simulink model "normal"  (R2020a)
settings: Solver=ode45  StartTime=0.0  StopTime=0.4  FixedStep=1e-6  MaxStep=0.04  RelTol=1e-3  EnableMultiTasking=on
PreLoadFcn:
  | power_13NodeTestFeeder_init;
values from neighbouring files (symbols this model uses):
  C_601 = [1.03835973183e-08  -3.28956213337e-09  -2.07596127216e-09; -3.28956213337e-09  9.8230300863e-09  -1.22250137004e-09; -2.07596127216e-09  -1.22250137004e-09  9.29377945947e-09]    [Finalmat.mat]    (also in bus1.mat; bus10.mat; bus11.mat; bus12.mat)
  C_602 = [9.39333329896e-09  -1.78290377777e-09  -2.78635373607e-09; -1.78290377777e-09  8.5370713848e-09  -1.08586207709e-09; -2.78635373607e-09  -1.08586207709e-09  8.94105559107e-09]    [Finalmat.mat]    (also in bus1.mat; bus10.mat; bus11.mat; bus12.mat)
  C_603 = [0  0  0; 0  7.76272711671e-09  -1.48325331387e-09; 0  -1.48325331387e-09  7.69036927641e-09]    [Finalmat.mat]    (also in bus1.mat; bus10.mat; bus11.mat; bus12.mat)
  C_604 = [7.69036927641e-09  0  -1.48325331387e-09; 0  0  0; -1.48325331387e-09  0  7.76272711671e-09]    [Finalmat.mat]    (also in bus1.mat; bus10.mat; bus11.mat; bus12.mat)
  C_605 = [0  0  0; 0  0  0; 0  0  7.44890176838e-09]    [Finalmat.mat]    (also in bus1.mat; bus10.mat; bus11.mat; bus12.mat)
  C_606 = [1.59697709306e-07  -1.64824237567e-15  -1.64824237567e-15; -1.64824237567e-15  1.59697709306e-07  -1.64824237567e-15; -1.64824237567e-15  -1.64824237567e-15  1.59697709306e-07]    [Finalmat.mat]    (also in bus1.mat; bus10.mat; bus11.mat; bus12.mat)
  C_607 = [1.46679066902e-07  0  0; 0  0  0; 0  0  0]    [Finalmat.mat]    (also in bus1.mat; bus10.mat; bus11.mat; bus12.mat)
  ft2km = 0.0003048    [Finalmat.mat]    (also in bus1.mat; bus10.mat; bus11.mat; bus12.mat)
  L_601 = [0.0016777459142  0.000826923199875  0.000698195470335; 0.000826923199875  0.00172702836123  0.000634408490396; 0.000698195470335  0.000634408490396  0.00170560121035]    [Finalmat.mat]    (also in bus1.mat; bus10.mat; bus11.mat; bus12.mat)
  L_602 = [0.00194723354262  0.000698195470335  0.000826923199875; 0.000698195470335  0.00197508883877  0.000634408490396; 0.000826923199875  0.000634408490396  0.00199635116541]    [Finalmat.mat]    (also in bus1.mat; bus10.mat; bus11.mat; bus12.mat)
  L_603 = [0  0  0; 0  0.00222034730427  0.000756708074671; 0  0.000756708074671  0.00223650007955]    [Finalmat.mat]    (also in bus1.mat; bus10.mat; bus11.mat; bus12.mat)
  L_604 = [0.00223650007955  0  0.000756708074671; 0  0  0; 0.000756708074671  0  0.00222034730427]    [Finalmat.mat]    (also in bus1.mat; bus10.mat; bus11.mat; bus12.mat)
  L_605 = [0  0  0; 0  0  0; 0  0  0.00222100660122]    [Finalmat.mat]    (also in bus1.mat; bus10.mat; bus11.mat; bus12.mat)
  L_606 = [0.000735610572263  5.40623499221e-05  2.35698659721e-05; 5.40623499221e-05  0.000666054744009  5.40623499221e-05; 2.35698659721e-05  5.40623499221e-05  0.000735610572263]    [Finalmat.mat]    (also in bus1.mat; bus10.mat; bus11.mat; bus12.mat)
  L_607 = [0.000844559393295  0  0; 0  0  0; 0  0  0]    [Finalmat.mat]    (also in bus1.mat; bus10.mat; bus11.mat; bus12.mat)
  R_601 = [0.215305653249  0.0969341469174  0.0981768923907; 0.0969341469174  0.209713298619  0.0953807150757; 0.0981768923907  0.0953807150757  0.212136652292]    [Finalmat.mat]    (also in bus1.mat; bus10.mat; bus11.mat; bus12.mat)
  R_602 = [0.467645121603  0.0981768923907  0.0969341469174; 0.0981768923907  0.464476120646  0.0953807150757; 0.0969341469174  0.0953807150757  0.462052766973]    [Finalmat.mat]    (also in bus1.mat; bus10.mat; bus11.mat; bus12.mat)
  R_603 = [0  0  0; 0  0.826052916102  0.128375607392; 0  0.128375607392  0.822573228777]    [Finalmat.mat]    (also in bus1.mat; bus10.mat; bus11.mat; bus12.mat)
  R_604 = [0.822573228777  0  0.128375607392; 0  0  0; 0.128375607392  0  0.826052916102]    [Finalmat.mat]    (also in bus1.mat; bus10.mat; bus11.mat; bus12.mat)
  R_605 = [0  0  0; 0  0  0; 0  0  0.825928641555]    [Finalmat.mat]    (also in bus1.mat; bus10.mat; bus11.mat; bus12.mat)
  R_606 = [0.495979718394  0.198342177539  0.177029092672; 0.198342177539  0.49032522649  0.198342177539; 0.177029092672  0.198342177539  0.495979718394]    [Finalmat.mat]    (also in bus1.mat; bus10.mat; bus11.mat; bus12.mat)
  R_607 = [0.834192898952  0  0; 0  0  0; 0  0  0]    [Finalmat.mat]    (also in bus1.mat; bus10.mat; bus11.mat; bus12.mat)
libraries: neural x322, powerlib x54, powerlib_meascontrol x6, simulink x1
(part 2 of 8)

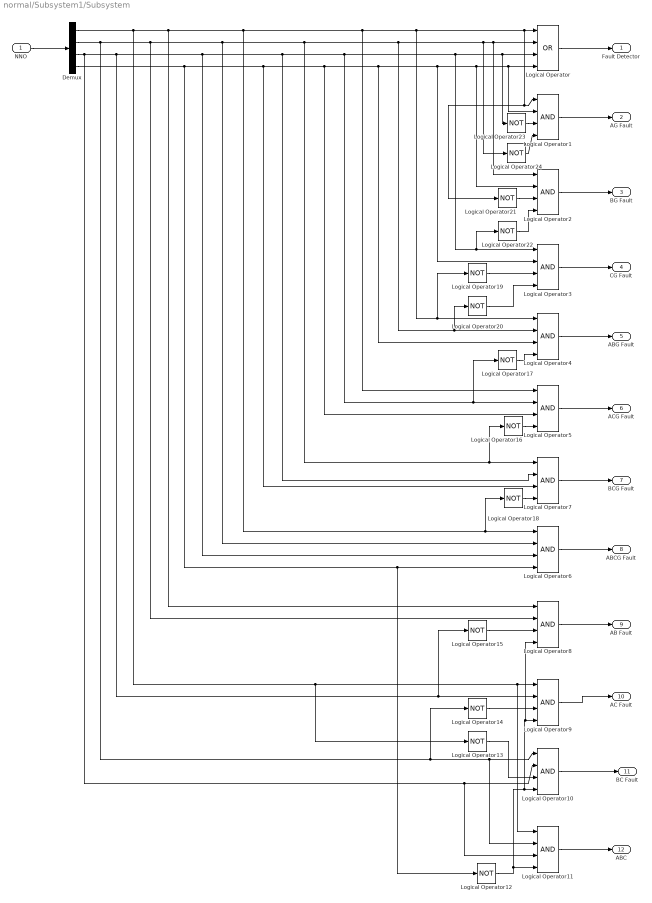
== system normal/Subsystem1/Subsystem ==
  NNO : Inport
  Demux : Demux
  Logical Operator : Logic  Operator=OR  Inputs=4  AllPortsSameDT=off  OutDataTypeStr=boolean
  Logical Operator{1..11} (11 alike) : Logic  Inputs=4  AllPortsSameDT=off  OutDataTypeStr=boolean
  Logical Operator{12..24} (13 alike) : Logic  Operator=NOT  AllPortsSameDT=off  OutDataTypeStr=boolean
  Fault Detector : Outport  VectorParamsAs1DForOutWhenUnconnected=off
  AG Fault : Outport  Port=2  VectorParamsAs1DForOutWhenUnconnected=off
  BG Fault : Outport  Port=3  VectorParamsAs1DForOutWhenUnconnected=off
  CG Fault : Outport  Port=4  VectorParamsAs1DForOutWhenUnconnected=off
  ABG Fault : Outport  Port=5  VectorParamsAs1DForOutWhenUnconnected=off
  ACG Fault : Outport  Port=6  VectorParamsAs1DForOutWhenUnconnected=off
  BCG Fault : Outport  Port=7  VectorParamsAs1DForOutWhenUnconnected=off
  ABCG Fault : Outport  Port=8  VectorParamsAs1DForOutWhenUnconnected=off
  AB Fault : Outport  Port=9  VectorParamsAs1DForOutWhenUnconnected=off
  AC Fault : Outport  Port=10  VectorParamsAs1DForOutWhenUnconnected=off
  BC Fault : Outport  Port=11  VectorParamsAs1DForOutWhenUnconnected=off
  ABC : Outport  Port=12  VectorParamsAs1DForOutWhenUnconnected=off
  wires:
  Logical Operator/1 -> Fault Detector/1
  NNO/1 -> Demux/1
  Demux/3 -> Logical Operator23/1, Logical Operator/3, Logical Operator22/1, Logical Operator3/1, Logical Operator17/1, Logical Operator5/2, Logical Operator7/2, Logical Operator6/3, Logical Operator15/1, Logical Operator9/2, Logical Operator11/3, Logical Operator10/2
  Demux/2 -> Logical Operator24/1, Logical Operator/2, Logical Operator2/1, Logical Operator20/1, Logical Operator4/2, Logical Operator16/1, Logical Operator7/1, Logical Operator6/2, Logical Operator8/2, Logical Operator14/1, Logical Operator11/2, Logical Operator10/1
  Demux/1 -> Logical Operator21/1, Logical Operator1/1, Logical Operator/1, Logical Operator19/1, Logical Operator4/1, Logical Operator5/1, Logical Operator18/1, Logical Operator6/1, Logical Operator8/1, Logical Operator13/1, Logical Operator11/1, Logical Operator9/1
  Demux/4 -> Logical Operator/4, Logical Operator1/2, Logical Operator2/2, Logical Operator3/2, Logical Operator4/3, Logical Operator5/3, Logical Operator7/3, Logical Operator12/1, Logical Operator6/4
  Logical Operator1/1 -> AG Fault/1
  Logical Operator2/1 -> BG Fault/1
  Logical Operator3/1 -> CG Fault/1
  Logical Operator4/1 -> ABG Fault/1
  Logical Operator5/1 -> ACG Fault/1
  Logical Operator7/1 -> BCG Fault/1
  Logical Operator6/1 -> ABCG Fault/1
  Logical Operator8/1 -> AB Fault/1
  Logical Operator11/1 -> ABC/1
  Logical Operator9/1 -> AC Fault/1
  Logical Operator10/1 -> BC Fault/1
  Logical Operator12/1 -> Logical Operator8/4, Logical Operator9/4, Logical Operator10/4, Logical Operator11/4
  Logical Operator13/1 -> Logical Operator10/3
  Logical Operator14/1 -> Logical Operator9/3
  Logical Operator15/1 -> Logical Operator8/3
  Logical Operator16/1 -> Logical Operator5/4
  Logical Operator17/1 -> Logical Operator4/4
  Logical Operator18/1 -> Logical Operator7/4
  Logical Operator19/1 -> Logical Operator3/3
  Logical Operator20/1 -> Logical Operator3/4
  Logical Operator22/1 -> Logical Operator2/4
  Logical Operator21/1 -> Logical Operator2/3
  Logical Operator23/1 -> Logical Operator1/3
  Logical Operator24/1 -> Logical Operator1/4

== system normal/Subsystem1/Function Fitting Neural Network/Layer 1 ==
  "p{1}" : Inport  PortDimensions=9
      mask Display: e = 0.06;c1 = [120 230 180]/255;c2 = ([120 230 180]+0)/(256+128);c3 = ([120 230 180]+128)/(256+128);patch([0 1 1 0],[0 0 1 1],c1);patch([0 1 1 1-e 1-e 0+e],[0 0 1 1-e 0+e 0+e],c2);patch([0 0 1 1-e 0+e 0+e],[0 1 1 1-e 1-e 0+e],c3);plot([0 1 1 0 0],[0 0 1 1 0]);
  Delays 1 : Subsystem
      mask Display: e = 0.06;c1 = [120 150 230]/255;c2 = ([120 150 230]+0)/383;c3 = ([120 150 230]+128)/383;patch([0 1 1 0],[0 0 1 1],c1);patch([0 1 1 1-e 1-e 0+e],[0 0 1 1-e 0+e 0+e],c2);patch([0 0 1 1-e 0+e 0+e],[0 1 1 1-e 1-e 0+e],c3);plot([0 1 1 0 0],[0 0 1 1 0]);disp('0');
  "IW{1,1}" : Subsystem
      mask Display: e = 0.06;c1 = [120 150 230]/255;c2 = ([120 150 230]+0)/383;c3 = ([120 150 230]+128)/383;patch([0 1 1 0],[0 0 1 1],c1);patch([0 1 1 1-e 1-e 0+e],[0 0 1 1-e 0+e 0+e],c2);patch([0 0 1 1-e 0+e 0+e],[0 1 1 1-e 1-e 0+e],c3);plot([0 1 1 0 0],[0 0 1 1 0]);disp('W');
  "b{1}" : Constant  Value=[1.4836701472282800562396687382715754210948944091796875;-4.6362530895366180772043662727810442447662353515625;-2.263086429812827926610907525173388421535491943359375;-2.5111547747930824669992944109253585338592529296875;0.56155923627202886105891366241849027574062347412109375;1.0307087915031150071598631257074885070323944091796875;-2.0460695401025663642258223262615501880645751953125;2.198522686181526797355445523862726986408233642578125;3.139278861361955552666813673567958176136016845703125;-1.9377980756718702348706528937327675521373748779296875;1.93447975728411147855467788758687674999237060546875;-1.9964334154407457067037512388196773827075958251953125;1.811849934043773036052016323083080351352691650390625;6.35238326894225480145905748941004276275634765625;3.1235450167660996356744362856261432170867919921875;-1.443640549170277953550112215452827513217926025390625;1.903051229366258478847839796799235045909881591796875;1.4333494363031633600513714554836042225360870361328125;-1.7974223905719768357158727667410857975482940673828125;-1.3000791505200501863015460912720300257205963134765625;0.392746284772382381333954981528222560882568359375;-1.78500042653535739844983254442922770977020263671875;1.5169851828956930628322652410133741796016693115234375;1.3899196529326232063539237060467712581157684326171875;0.88142263857842573226974991484894417226314544677734375;1.1298077443202012570822034831508062779903411865234375;1.6602576721865756059770546926301904022693634033203125;1.223520547142563419384941880707629024982452392578125;-1.520268524491023232059205838595516979694366455078125;0.929306052241560820448285085149109363555908203125;0.7195182400574877679133578567416407167911529541015625;0.53584680856447641783546487204148434102535247802734375;-2.402562935457116299886592969414778053760528564453125;0.0090962459951229000798544888084506965242326259613037109375;3.78523511409148749606856654281727969646453857421875;-0.14178662349532833442111723343259654939174652099609375;-0.34916324318866764908619870766415260732173919677734375;-0.42829990541065343645499297053902409970760345458984375;1.0935762893525506900260779730160720646381378173828125;0.7933443401718462961724753768066875636577606201171875;-0.19596363861845167431141589986509643495082855224609375;-2.881071814469615244291844646795652806758880615234375;2.561797995207929279359859719988889992237091064453125;-0.54218651761972835867453568425844423472881317138671875;-2.65640312734315831022513521020300686359405517578125;0.446493577723002743606883768734405748546123504638671875;-0.17177045244666844237002578665851615369319915771484375;-0.45537132588368745000906301356735639274120330810546875;-0.295732407345984660285154177472577430307865142822265625;-0.7946266943011830452547883396618999540805816650390625;0.9019892031651222108479259986779652535915374755859375;-0.5924118385813235132530962800956331193447113037109375;0.8851509988800858597102205749251879751682281494140625;-1.032020499483159436948653819854371249675750732421875;0.048154807323418695463868033357357489876449108123779296875;-0.72862529927491959114149722154252231121063232421875;0.9210456908434763168003200917155481874942779541015625;-2.14382668683358534877925194450654089450836181640625;0.128247662536615181227972470878739841282367706298828125;0.7914028966542192566890889793285168707370758056640625;-2.100152108028215724999654412386007606983184814453125;-0.075866072480479385120588631252758204936981201171875;0.2336366489054485795495708089219988323748111724853515625;2.12112491398540026210639553028158843517303466796875;-0.64362822141550546373167662750347517430782318115234375;0.9649124469060008646437154311570338904857635498046875;-0.85346406017299869528613953661988489329814910888671875;-0.47601133976015630455691507449955679476261138916015625;0.2488827845882790879006307704912615008652210235595703125;-0.10602051256760088027153443590577808208763599395751953125;2.0229387007712755774946344899944961071014404296875;0.8915126324932642898346557558397762477397918701171875 ...(+1511 chars)]
      mask Display: e = 0.06;c1 = [120 150 230]/255;c2 = ([120 150 230]+0)/383;c3 = ([120 150 230]+128)/383;patch([0 1 1 0],[0 0 1 1],c1);patch([0 1 1 1-e 1-e 0+e],[0 0 1 1-e 0+e 0+e],c2);patch([0 0 1 1-e 0+e 0+e],[0 1 1 1-e 1-e 0+e],c3);plot([0 1 1 0 0],[0 0 1 1 0]);disp('b');
  netsum : Sum  Inputs=2  InputSameDT=on  SaturateOnIntegerOverflow=on  OutDataTypeStr=Inherit: Same as first input
      mask Display: e = 0.06;c1 = [120 150 230]/255;c2 = ([120 150 230]+0)/383;c3 = ([120 150 230]+128)/383;patch([0 1 1 0],[0 0 1 1],c1);patch([0 1 1 1-e 1-e 0+e],[0 0 1 1-e 0+e 0+e],c2);patch([0 0 1 1-e 0+e 0+e],[0 1 1 1-e 1-e 0+e],c3);plot([0 1 1 0 0],[0 0 1 1 0]);disp('+');
  tansig : neural/Transfer Functions/tansig
  "a{1}" : Outport  InitialOutput=[0;0;0;0;0;0;0;0;0;0;0;0;0;0;0;0;0;0;0;0;0;0;0;0;0;0;0;0;0;0;0;0;0;0;0;0;0;0;0;0;0;0;0;0;0;0;0;0;0;0;0;0;0;0;0;0;0;0;0;0;0;0;0;0;0;0;0;0;0;0;0;0;0;0;0;0;0;0;0;0;0;0;0;0;0;0;0;0;0;0;0;0;0;0;0;0;0;0;0;0]
      mask Display: e = 0.06;c1 = [120 230 180]/255;c2 = ([120 230 180]+0)/(256+128);c3 = ([120 230 180]+128)/(256+128);patch([0 1 1 0],[0 0 1 1],c1);patch([0 1 1 1-e 1-e 0+e],[0 0 1 1-e 0+e 0+e],c2);patch([0 0 1 1-e 0+e 0+e],[0 1 1 1-e 1-e 0+e],c3);plot([0 1 1 0 0],[0 0 1 1 0]);
  wires:
  "p{1}"/1 -> Delays 1/1("p{1}")
  Delays 1/1("pd{1,1}") -> "IW{1,1}"/1("pd{1,1}")
  "IW{1,1}"/1("iz{1,1}") -> netsum/1
  "b{1}"/1 -> netsum/2
  netsum/1 -> tansig/1
  tansig/1 -> "a{1}"/1

== system normal/Subsystem1/Function Fitting Neural Network/Layer 2 ==
  "a{1} " : Inport  PortDimensions=100
      mask Display: e = 0.06;c1 = [120 230 180]/255;c2 = ([120 230 180]+0)/(256+128);c3 = ([120 230 180]+128)/(256+128);patch([0 1 1 0],[0 0 1 1],c1);patch([0 1 1 1-e 1-e 0+e],[0 0 1 1-e 0+e 0+e],c2);patch([0 0 1 1-e 0+e 0+e],[0 1 1 1-e 1-e 0+e],c3);plot([0 1 1 0 0],[0 0 1 1 0]);
  Delays 1 : Subsystem
      mask Display: e = 0.06;c1 = [120 150 230]/255;c2 = ([120 150 230]+0)/383;c3 = ([120 150 230]+128)/383;patch([0 1 1 0],[0 0 1 1],c1);patch([0 1 1 1-e 1-e 0+e],[0 0 1 1-e 0+e 0+e],c2);patch([0 0 1 1-e 0+e 0+e],[0 1 1 1-e 1-e 0+e],c3);plot([0 1 1 0 0],[0 0 1 1 0]);disp('0');
  "LW{2,1}" : Subsystem
      mask Display: e = 0.06;c1 = [120 150 230]/255;c2 = ([120 150 230]+0)/383;c3 = ([120 150 230]+128)/383;patch([0 1 1 0],[0 0 1 1],c1);patch([0 1 1 1-e 1-e 0+e],[0 0 1 1-e 0+e 0+e],c2);patch([0 0 1 1-e 0+e 0+e],[0 1 1 1-e 1-e 0+e],c3);plot([0 1 1 0 0],[0 0 1 1 0]);disp('W');
  "b{2}" : Constant  Value=0.73666496147771398650405672015040181577205657958984375
      mask Display: e = 0.06;c1 = [120 150 230]/255;c2 = ([120 150 230]+0)/383;c3 = ([120 150 230]+128)/383;patch([0 1 1 0],[0 0 1 1],c1);patch([0 1 1 1-e 1-e 0+e],[0 0 1 1-e 0+e 0+e],c2);patch([0 0 1 1-e 0+e 0+e],[0 1 1 1-e 1-e 0+e],c3);plot([0 1 1 0 0],[0 0 1 1 0]);disp('b');
  netsum : Sum  Inputs=2  InputSameDT=on  SaturateOnIntegerOverflow=on  OutDataTypeStr=Inherit: Same as first input
      mask Display: e = 0.06;c1 = [120 150 230]/255;c2 = ([120 150 230]+0)/383;c3 = ([120 150 230]+128)/383;patch([0 1 1 0],[0 0 1 1],c1);patch([0 1 1 1-e 1-e 0+e],[0 0 1 1-e 0+e 0+e],c2);patch([0 0 1 1-e 0+e 0+e],[0 1 1 1-e 1-e 0+e],c3);plot([0 1 1 0 0],[0 0 1 1 0]);disp('+');
  purelin : neural/Transfer Functions/purelin
  "a{2}" : Outport  InitialOutput=0
      mask Display: e = 0.06;c1 = [120 230 180]/255;c2 = ([120 230 180]+0)/(256+128);c3 = ([120 230 180]+128)/(256+128);patch([0 1 1 0],[0 0 1 1],c1);patch([0 1 1 1-e 1-e 0+e],[0 0 1 1-e 0+e 0+e],c2);patch([0 0 1 1-e 0+e 0+e],[0 1 1 1-e 1-e 0+e],c3);plot([0 1 1 0 0],[0 0 1 1 0]);
  wires:
  "a{1} "/1 -> Delays 1/1("p{2}")
  Delays 1/1("pd{2,1}") -> "LW{2,1}"/1("ad{2,1}")
  "LW{2,1}"/1("lz{2,1}") -> netsum/1
  "b{2}"/1 -> netsum/2
  netsum/1 -> purelin/1
  purelin/1 -> "a{2}"/1

== system normal/Subsystem1/Function Fitting Neural Network/Process Input 1 ==
  x : Inport  PortDimensions=9
      mask Display: e = 0.06;c1 = [120 230 180]/255;c2 = ([120 230 180]+0)/(256+128);c3 = ([120 230 180]+128)/(256+128);patch([0 1 1 0],[0 0 1 1],c1);patch([0 1 1 1-e 1-e 0+e],[0 0 1 1-e 0+e 0+e],c2);patch([0 0 1 1-e 0+e 0+e],[0 1 1 1-e 1-e 0+e],c3);plot([0 1 1 0 0],[0 0 1 1 0]);
  mapminmax : neural/Processing Functions/mapminmax  xmin=[4.0361303012440723492204597278;2.7248060221038734596277208766;4.10876986009723044190877772053;11.7997395123970481023434331291;9.69147739713131528560552396812;3.46457612151836746861022220401;6.39593571872652155718697031261;4.28688363604756350611069137813;6.97687974683904688077973332838]  xmax=[1771.43499266887192788999527693;1794.0488976631054356403183192;1779.62314843343483516946434975;2484.57589134188310708850622177;2501.74066788909203751245513558;2464.12499617464936818578280509;15623.5974818944614526117220521;15525.5512130097831686725839972;13147.2305966597232327330857515]  ymin=-1  ymax=1
  p : Outport  PortDimensions=9
      mask Display: e = 0.06;c1 = [120 230 180]/255;c2 = ([120 230 180]+0)/(256+128);c3 = ([120 230 180]+128)/(256+128);patch([0 1 1 0],[0 0 1 1],c1);patch([0 1 1 1-e 1-e 0+e],[0 0 1 1-e 0+e 0+e],c2);patch([0 0 1 1-e 0+e 0+e],[0 1 1 1-e 1-e 0+e],c3);plot([0 1 1 0 0],[0 0 1 1 0]);
  wires:
  x/1 -> mapminmax/1
  mapminmax/1 -> p/1

== system normal/Subsystem1/Function Fitting Neural Network/Process Output 1 ==
  a : Inport  PortDimensions=1
      mask Display: e = 0.06;c1 = [120 230 180]/255;c2 = ([120 230 180]+0)/(256+128);c3 = ([120 230 180]+128)/(256+128);patch([0 1 1 0],[0 0 1 1],c1);patch([0 1 1 1-e 1-e 0+e],[0 0 1 1-e 0+e 0+e],c2);patch([0 0 1 1-e 0+e 0+e],[0 1 1 1-e 1-e 0+e],c3);plot([0 1 1 0 0],[0 0 1 1 0]);
  mapminmax_reverse : neural/Processing Functions/mapminmax_reverse  xmin=0  xmax=6920  ymin=-1  ymax=1
  y : Outport  PortDimensions=1
      mask Display: e = 0.06;c1 = [120 230 180]/255;c2 = ([120 230 180]+0)/(256+128);c3 = ([120 230 180]+128)/(256+128);patch([0 1 1 0],[0 0 1 1],c1);patch([0 1 1 1-e 1-e 0+e],[0 0 1 1-e 0+e 0+e],c2);patch([0 0 1 1-e 0+e 0+e],[0 1 1 1-e 1-e 0+e],c3);plot([0 1 1 0 0],[0 0 1 1 0]);
  wires:
  a/1 -> mapminmax_reverse/1
  mapminmax_reverse/1 -> y/1

== system normal/Subsystem1/Function Fitting Neural Network1/Layer 1 ==
  "p{1}" : Inport  PortDimensions=9
      mask Display: e = 0.06;c1 = [120 230 180]/255;c2 = ([120 230 180]+0)/(256+128);c3 = ([120 230 180]+128)/(256+128);patch([0 1 1 0],[0 0 1 1],c1);patch([0 1 1 1-e 1-e 0+e],[0 0 1 1-e 0+e 0+e],c2);patch([0 0 1 1-e 0+e 0+e],[0 1 1 1-e 1-e 0+e],c3);plot([0 1 1 0 0],[0 0 1 1 0]);
  Delays 1 : Subsystem
      mask Display: e = 0.06;c1 = [120 150 230]/255;c2 = ([120 150 230]+0)/383;c3 = ([120 150 230]+128)/383;patch([0 1 1 0],[0 0 1 1],c1);patch([0 1 1 1-e 1-e 0+e],[0 0 1 1-e 0+e 0+e],c2);patch([0 0 1 1-e 0+e 0+e],[0 1 1 1-e 1-e 0+e],c3);plot([0 1 1 0 0],[0 0 1 1 0]);disp('0');
  "IW{1,1}" : Subsystem
      mask Display: e = 0.06;c1 = [120 150 230]/255;c2 = ([120 150 230]+0)/383;c3 = ([120 150 230]+128)/383;patch([0 1 1 0],[0 0 1 1],c1);patch([0 1 1 1-e 1-e 0+e],[0 0 1 1-e 0+e 0+e],c2);patch([0 0 1 1-e 0+e 0+e],[0 1 1 1-e 1-e 0+e],c3);plot([0 1 1 0 0],[0 0 1 1 0]);disp('W');
  "b{1}" : Constant  Value=[-2.13037715805268224045221359119750559329986572265625;2.746628097332809215203042185748927295207977294921875;2.796820994036730123610823284252546727657318115234375;0.4379379172983457468859569416963495314121246337890625;3.19223672506301081597257507382892072200775146484375;2.32496861654698694366061317850835621356964111328125;4.96726265985274917369451941340230405330657958984375;-1.697889576240742659507532152929343283176422119140625;2.298342309252483506298858628724701702594757080078125;1.966788681545197814415359971462748944759368896484375;-1.6125818559296110077383445968735031783580780029296875;1.5932178234269305239223513126489706337451934814453125;2.128810638902830731922222184948623180389404296875;-1.8112450514425881831215292550041340291500091552734375;-1.5788526096734150083733538849628530442714691162109375;-1.7955601924814892367265883876825682818889617919921875;-1.5849459381517727596389022437506355345249176025390625;-1.239288634212896145214699572534300386905670166015625;1.7228555051975666945196508095250464975833892822265625;-1.91686706005321649826100838254205882549285888671875;1.136660428733942129753131666802801191806793212890625;1.6784310129253030563489801352261565625667572021484375;-1.2868677081393820049726173238013871014118194580078125;1.4370556408635486445035667202319018542766571044921875;-1.5666891013466555104827193645178340375423431396484375;0.9782525744571939352312028859159909188747406005859375;1.56716358617225726135302465991117060184478759765625;-1.6998176443286594494708197089494206011295318603515625;-1.5458464297808092169361771084368228912353515625;1.0272554098359225616121648272383026778697967529296875;-1.1686228030247203246716480862232856452465057373046875;1.2392503600146891340472166120889596641063690185546875;-1.189381954438957667008480711956508457660675048828125;0.75198983869119218059751119653810746967792510986328125;0.358705656692439978083797313956893049180507659912109375;-0.92787680539037664662060933551401831209659576416015625;0.92975961512061078284574477947899140417575836181640625;-1.6601127850120409590317649417556822299957275390625;0.6862163993559653452081192881450988352298736572265625;0.351615586023979964647168117153341881930828094482421875;-0.9718618814417145923556518027908168733119964599609375;0.3834890515686317780108538499916903674602508544921875;1.1866027668763285962683085017488338053226470947265625;0.1954793823718590506377523752234992571175098419189453125;9.717970888699387188580658403225243091583251953125;5.33150149385156968406818123185075819492340087890625;0.47179814055236024561423846535035409033298492431640625;1.04948464890701931295780013897456228733062744140625;-0.95703425531130914549748922581784427165985107421875;0.1182206558537874097059017231003963388502597808837890625;0.150928108369996094584308821140439249575138092041015625;1.4935520252605691826630618379567749798297882080078125;-0.1574597910620717244878363771931617520749568939208984375;-0.493842571590737244857649557161494158208370208740234375;-0.1422139229762254541977739563662908039987087249755859375;-1.1294062657578962660664956274558790028095245361328125;6.2652904988000432950911999796517193317413330078125;-0.165122232426719417475169393583200871944427490234375;-0.7390589492982815311705735439318232238292694091796875;2.2778886380741969475138830603100359439849853515625;-0.2308917333994849607758936826940043829381465911865234375;0.171927231209594688632336101363762281835079193115234375;-0.69931808506733739161376206538989208638668060302734375;-0.43528701845326567276828200192539952695369720458984375;-1.708972287139544743439500962267629802227020263671875;-1.1665184635571332893988483192515559494495391845703125;1.14387762923370939205369722913019359111785888671875;1.48052201410643835544078683597035706043243408203125;-2.107332378231126401857409291551448404788970947265625;-3.493579865692837405077852963586337864398956298828125;1.414814221395528814895214964053593575954437255859375;0.06447901910621141319257532131814514286816120147705078125 ...(+1519 chars)]
      mask Display: e = 0.06;c1 = [120 150 230]/255;c2 = ([120 150 230]+0)/383;c3 = ([120 150 230]+128)/383;patch([0 1 1 0],[0 0 1 1],c1);patch([0 1 1 1-e 1-e 0+e],[0 0 1 1-e 0+e 0+e],c2);patch([0 0 1 1-e 0+e 0+e],[0 1 1 1-e 1-e 0+e],c3);plot([0 1 1 0 0],[0 0 1 1 0]);disp('b');
  netsum : Sum  Inputs=2  InputSameDT=on  SaturateOnIntegerOverflow=on  OutDataTypeStr=Inherit: Same as first input
      mask Display: e = 0.06;c1 = [120 150 230]/255;c2 = ([120 150 230]+0)/383;c3 = ([120 150 230]+128)/383;patch([0 1 1 0],[0 0 1 1],c1);patch([0 1 1 1-e 1-e 0+e],[0 0 1 1-e 0+e 0+e],c2);patch([0 0 1 1-e 0+e 0+e],[0 1 1 1-e 1-e 0+e],c3);plot([0 1 1 0 0],[0 0 1 1 0]);disp('+');
  tansig : neural/Transfer Functions/tansig
  "a{1}" : Outport  InitialOutput=[0;0;0;0;0;0;0;0;0;0;0;0;0;0;0;0;0;0;0;0;0;0;0;0;0;0;0;0;0;0;0;0;0;0;0;0;0;0;0;0;0;0;0;0;0;0;0;0;0;0;0;0;0;0;0;0;0;0;0;0;0;0;0;0;0;0;0;0;0;0;0;0;0;0;0;0;0;0;0;0;0;0;0;0;0;0;0;0;0;0;0;0;0;0;0;0;0;0;0;0]
      mask Display: e = 0.06;c1 = [120 230 180]/255;c2 = ([120 230 180]+0)/(256+128);c3 = ([120 230 180]+128)/(256+128);patch([0 1 1 0],[0 0 1 1],c1);patch([0 1 1 1-e 1-e 0+e],[0 0 1 1-e 0+e 0+e],c2);patch([0 0 1 1-e 0+e 0+e],[0 1 1 1-e 1-e 0+e],c3);plot([0 1 1 0 0],[0 0 1 1 0]);
  wires:
  "p{1}"/1 -> Delays 1/1("p{1}")
  Delays 1/1("pd{1,1}") -> "IW{1,1}"/1("pd{1,1}")
  "IW{1,1}"/1("iz{1,1}") -> netsum/1
  "b{1}"/1 -> netsum/2
  netsum/1 -> tansig/1
  tansig/1 -> "a{1}"/1

== system normal/Subsystem1/Function Fitting Neural Network1/Layer 2 ==
  "a{1} " : Inport  PortDimensions=100
      mask Display: e = 0.06;c1 = [120 230 180]/255;c2 = ([120 230 180]+0)/(256+128);c3 = ([120 230 180]+128)/(256+128);patch([0 1 1 0],[0 0 1 1],c1);patch([0 1 1 1-e 1-e 0+e],[0 0 1 1-e 0+e 0+e],c2);patch([0 0 1 1-e 0+e 0+e],[0 1 1 1-e 1-e 0+e],c3);plot([0 1 1 0 0],[0 0 1 1 0]);
  Delays 1 : Subsystem
      mask Display: e = 0.06;c1 = [120 150 230]/255;c2 = ([120 150 230]+0)/383;c3 = ([120 150 230]+128)/383;patch([0 1 1 0],[0 0 1 1],c1);patch([0 1 1 1-e 1-e 0+e],[0 0 1 1-e 0+e 0+e],c2);patch([0 0 1 1-e 0+e 0+e],[0 1 1 1-e 1-e 0+e],c3);plot([0 1 1 0 0],[0 0 1 1 0]);disp('0');
  "LW{2,1}" : Subsystem
      mask Display: e = 0.06;c1 = [120 150 230]/255;c2 = ([120 150 230]+0)/383;c3 = ([120 150 230]+128)/383;patch([0 1 1 0],[0 0 1 1],c1);patch([0 1 1 1-e 1-e 0+e],[0 0 1 1-e 0+e 0+e],c2);patch([0 0 1 1-e 0+e 0+e],[0 1 1 1-e 1-e 0+e],c3);plot([0 1 1 0 0],[0 0 1 1 0]);disp('W');
  "b{2}" : Constant  Value=[-0.276103633206194298832514277819427661597728729248046875;-0.592478370382765628932020263164304196834564208984375;1.21968178273867788874440520885400474071502685546875;1.6162405288693333371696780886850319802761077880859375]
      mask Display: e = 0.06;c1 = [120 150 230]/255;c2 = ([120 150 230]+0)/383;c3 = ([120 150 230]+128)/383;patch([0 1 1 0],[0 0 1 1],c1);patch([0 1 1 1-e 1-e 0+e],[0 0 1 1-e 0+e 0+e],c2);patch([0 0 1 1-e 0+e 0+e],[0 1 1 1-e 1-e 0+e],c3);plot([0 1 1 0 0],[0 0 1 1 0]);disp('b');
  netsum : Sum  Inputs=2  InputSameDT=on  SaturateOnIntegerOverflow=on  OutDataTypeStr=Inherit: Same as first input
      mask Display: e = 0.06;c1 = [120 150 230]/255;c2 = ([120 150 230]+0)/383;c3 = ([120 150 230]+128)/383;patch([0 1 1 0],[0 0 1 1],c1);patch([0 1 1 1-e 1-e 0+e],[0 0 1 1-e 0+e 0+e],c2);patch([0 0 1 1-e 0+e 0+e],[0 1 1 1-e 1-e 0+e],c3);plot([0 1 1 0 0],[0 0 1 1 0]);disp('+');
  purelin : neural/Transfer Functions/purelin
  "a{2}" : Outport  InitialOutput=[0;0;0;0]
      mask Display: e = 0.06;c1 = [120 230 180]/255;c2 = ([120 230 180]+0)/(256+128);c3 = ([120 230 180]+128)/(256+128);patch([0 1 1 0],[0 0 1 1],c1);patch([0 1 1 1-e 1-e 0+e],[0 0 1 1-e 0+e 0+e],c2);patch([0 0 1 1-e 0+e 0+e],[0 1 1 1-e 1-e 0+e],c3);plot([0 1 1 0 0],[0 0 1 1 0]);
  wires:
  "a{1} "/1 -> Delays 1/1("p{2}")
  Delays 1/1("pd{2,1}") -> "LW{2,1}"/1("ad{2,1}")
  "LW{2,1}"/1("lz{2,1}") -> netsum/1
  "b{2}"/1 -> netsum/2
  netsum/1 -> purelin/1
  purelin/1 -> "a{2}"/1

== system normal/Subsystem1/Function Fitting Neural Network1/Process Input 1 ==
  x : Inport  PortDimensions=9
      mask Display: e = 0.06;c1 = [120 230 180]/255;c2 = ([120 230 180]+0)/(256+128);c3 = ([120 230 180]+128)/(256+128);patch([0 1 1 0],[0 0 1 1],c1);patch([0 1 1 1-e 1-e 0+e],[0 0 1 1-e 0+e 0+e],c2);patch([0 0 1 1-e 0+e 0+e],[0 1 1 1-e 1-e 0+e],c3);plot([0 1 1 0 0],[0 0 1 1 0]);
  mapminmax : neural/Processing Functions/mapminmax  xmin=[4.0361303012440723492204597278;2.7248060221038734596277208766;4.10876986009723044190877772053;11.7997395123970481023434331291;9.69147739713131528560552396812;3.46457612151836746861022220401;6.39593571872652155718697031261;4.28688363604756350611069137813;6.97687974683904688077973332838]  xmax=[1771.43499266887192788999527693;1794.0488976631054356403183192;1779.62314843343483516946434975;2484.57589134188310708850622177;2501.74066788909203751245513558;2464.12499617464936818578280509;15623.5974818944614526117220521;15525.5512130097831686725839972;13147.2305966597232327330857515]  ymin=-1  ymax=1
  p : Outport  PortDimensions=9
      mask Display: e = 0.06;c1 = [120 230 180]/255;c2 = ([120 230 180]+0)/(256+128);c3 = ([120 230 180]+128)/(256+128);patch([0 1 1 0],[0 0 1 1],c1);patch([0 1 1 1-e 1-e 0+e],[0 0 1 1-e 0+e 0+e],c2);patch([0 0 1 1-e 0+e 0+e],[0 1 1 1-e 1-e 0+e],c3);plot([0 1 1 0 0],[0 0 1 1 0]);
  wires:
  x/1 -> mapminmax/1
  mapminmax/1 -> p/1

== system normal/Subsystem1/Function Fitting Neural Network1/Process Output 1 ==
  a : Inport  PortDimensions=4
      mask Display: e = 0.06;c1 = [120 230 180]/255;c2 = ([120 230 180]+0)/(256+128);c3 = ([120 230 180]+128)/(256+128);patch([0 1 1 0],[0 0 1 1],c1);patch([0 1 1 1-e 1-e 0+e],[0 0 1 1-e 0+e 0+e],c2);patch([0 0 1 1-e 0+e 0+e],[0 1 1 1-e 1-e 0+e],c3);plot([0 1 1 0 0],[0 0 1 1 0]);
  mapminmax_reverse : neural/Processing Functions/mapminmax_reverse  xmin=[0;0;0;0]  xmax=[1;1;1;1]  ymin=-1  ymax=1
  y : Outport  PortDimensions=4
      mask Display: e = 0.06;c1 = [120 230 180]/255;c2 = ([120 230 180]+0)/(256+128);c3 = ([120 230 180]+128)/(256+128);patch([0 1 1 0],[0 0 1 1],c1);patch([0 1 1 1-e 1-e 0+e],[0 0 1 1-e 0+e 0+e],c2);patch([0 0 1 1-e 0+e 0+e],[0 1 1 1-e 1-e 0+e],c3);plot([0 1 1 0 0],[0 0 1 1 0]);
  wires:
  a/1 -> mapminmax_reverse/1
  mapminmax_reverse/1 -> y/1

== system normal/Subsystem1/Function Fitting Neural Network2/Layer 1 ==
  "p{1}" : Inport  PortDimensions=13
      mask Display: e = 0.06;c1 = [120 230 180]/255;c2 = ([120 230 180]+0)/(256+128);c3 = ([120 230 180]+128)/(256+128);patch([0 1 1 0],[0 0 1 1],c1);patch([0 1 1 1-e 1-e 0+e],[0 0 1 1-e 0+e 0+e],c2);patch([0 0 1 1-e 0+e 0+e],[0 1 1 1-e 1-e 0+e],c3);plot([0 1 1 0 0],[0 0 1 1 0]);
  Delays 1 : Subsystem
      mask Display: e = 0.06;c1 = [120 150 230]/255;c2 = ([120 150 230]+0)/383;c3 = ([120 150 230]+128)/383;patch([0 1 1 0],[0 0 1 1],c1);patch([0 1 1 1-e 1-e 0+e],[0 0 1 1-e 0+e 0+e],c2);patch([0 0 1 1-e 0+e 0+e],[0 1 1 1-e 1-e 0+e],c3);plot([0 1 1 0 0],[0 0 1 1 0]);disp('0');
  "IW{1,1}" : Subsystem
      mask Display: e = 0.06;c1 = [120 150 230]/255;c2 = ([120 150 230]+0)/383;c3 = ([120 150 230]+128)/383;patch([0 1 1 0],[0 0 1 1],c1);patch([0 1 1 1-e 1-e 0+e],[0 0 1 1-e 0+e 0+e],c2);patch([0 0 1 1-e 0+e 0+e],[0 1 1 1-e 1-e 0+e],c3);plot([0 1 1 0 0],[0 0 1 1 0]);disp('W');
  "b{1}" : Constant  Value=[1.81395476471276761998296933597885072231292724609375;2.7194376942024991450352899846620857715606689453125;-1.72349860831830792307073352276347577571868896484375;-1.821116239033454764495445488137193024158477783203125;-1.93638771609739901435887077241204679012298583984375;2.06687310998890882984824202139861881732940673828125;-1.6673370286661228778513077486422844231128692626953125;-1.8370667948424623805436795009882189333438873291015625;2.14254149701795171267804107628762722015380859375;-1.6306345123111061212739514303393661975860595703125;1.16236256409761562480298380251042544841766357421875;1.5484167971076379100026088053709827363491058349609375;-1.48574282248885314317021766328252851963043212890625;-1.68619347385013185203206376172602176666259765625;-2.05039026135216584378895277041010558605194091796875;-0.328502713000412338573141823871992528438568115234375;1.9150886628088230612121378726442344486713409423828125;-1.360330567283977387660343083553016185760498046875;-2.129181993334120281957666520611383020877838134765625;-0.1312933934919937595253713880083523690700531005859375;4.85193313264938463902353760204277932643890380859375;-2.597198527519215094372384555754251778125762939453125;2.326984365054592718280446206335909664630889892578125;-1.006372015756110016582169919274747371673583984375;4.07414598448991061019341941573657095432281494140625;-0.7456033221682096812088502701953984797000885009765625;0.9742672808679804230536092291004024446010589599609375;0.78192000944506501181052726678899489343166351318359375;0.91816292040349833936119239297113381326198577880859375;0.70098744374508481502772383464616723358631134033203125;-0.49973563865602044220537436558515764772891998291015625;-0.34573755131770933513024601779761724174022674560546875;0.8827250866996643186013216109131462872028350830078125;0.90617648258656824378221017468604259192943572998046875;0.59274500128733276227421811199747025966644287109375;1.5834228568403820869292530915117822587490081787109375;0.394331646477629027547351370230899192392826080322265625;-0.82408218616843698089979852738906629383563995361328125;0.49612969826781505577883990554255433380603790283203125;-1.72935939154759221736412655445747077465057373046875;1.1232305293915396671167172826244495809078216552734375;-0.050110843549257426399190507027014973573386669158935546875;-0.81152116107212635132128752957214601337909698486328125;-2.07660546963558800825921935029327869415283203125;-1.3110962078801866592669966848916374146938323974609375;1.1979587506872528823720358559512533247470855712890625;-0.410077031084450982501010685155051760375499725341796875;-0.05351676262684408602599006599120912142097949981689453125;0.6183106422134141411106611485593020915985107421875;0.87083582382769808560851743095554411411285400390625;-0.53718685339921246058025872116559185087680816650390625;1.742109845522545885643239671480841934680938720703125;0.431754807586093136695382099787821061909198760986328125;1.4370914450336211842795819393359124660491943359375;0.16949321549061568958904899773187935352325439453125;0.575682169926941877946546810562722384929656982421875;0.6907107855324061684854086706764064729213714599609375;-0.63274195580283321138637120384373702108860015869140625;-1.1341959457971935165687682456336915493011474609375;0.4377308440451967985751480227918364107608795166015625;-0.256482446084123238971841374223004095256328582763671875;-3.24466252695743406775363837368786334991455078125;-0.525002886800031820513368074898608028888702392578125;-0.44844157027907083357121109656873159110546112060546875;-0.9633730537686648887074625235982239246368408203125;1.225647789665470721587325897417031228542327880859375;-0.382521412243540359643390047494904138147830963134765625;1.9681507228063976899790077368379570543766021728515625;-1.123532721125788835792036479688249528408050537109375;0.427041136588554248731952611706219613552093505859375;-0.34618128575157902648840035908506251871585845947265625;-1.4521058597778051524329612220753915607929229736328125;-0.8002175294299860297542181797325611114501953125 ...(+1462 chars)]
      mask Display: e = 0.06;c1 = [120 150 230]/255;c2 = ([120 150 230]+0)/383;c3 = ([120 150 230]+128)/383;patch([0 1 1 0],[0 0 1 1],c1);patch([0 1 1 1-e 1-e 0+e],[0 0 1 1-e 0+e 0+e],c2);patch([0 0 1 1-e 0+e 0+e],[0 1 1 1-e 1-e 0+e],c3);plot([0 1 1 0 0],[0 0 1 1 0]);disp('b');
  netsum : Sum  Inputs=2  InputSameDT=on  SaturateOnIntegerOverflow=on  OutDataTypeStr=Inherit: Same as first input
      mask Display: e = 0.06;c1 = [120 150 230]/255;c2 = ([120 150 230]+0)/383;c3 = ([120 150 230]+128)/383;patch([0 1 1 0],[0 0 1 1],c1);patch([0 1 1 1-e 1-e 0+e],[0 0 1 1-e 0+e 0+e],c2);patch([0 0 1 1-e 0+e 0+e],[0 1 1 1-e 1-e 0+e],c3);plot([0 1 1 0 0],[0 0 1 1 0]);disp('+');
  tansig : neural/Transfer Functions/tansig
  "a{1}" : Outport  InitialOutput=[0;0;0;0;0;0;0;0;0;0;0;0;0;0;0;0;0;0;0;0;0;0;0;0;0;0;0;0;0;0;0;0;0;0;0;0;0;0;0;0;0;0;0;0;0;0;0;0;0;0;0;0;0;0;0;0;0;0;0;0;0;0;0;0;0;0;0;0;0;0;0;0;0;0;0;0;0;0;0;0;0;0;0;0;0;0;0;0;0;0;0;0;0;0;0;0;0;0;0;0]
      mask Display: e = 0.06;c1 = [120 230 180]/255;c2 = ([120 230 180]+0)/(256+128);c3 = ([120 230 180]+128)/(256+128);patch([0 1 1 0],[0 0 1 1],c1);patch([0 1 1 1-e 1-e 0+e],[0 0 1 1-e 0+e 0+e],c2);patch([0 0 1 1-e 0+e 0+e],[0 1 1 1-e 1-e 0+e],c3);plot([0 1 1 0 0],[0 0 1 1 0]);
  wires:
  tansig/1 -> "a{1}"/1
  netsum/1 -> tansig/1
  "b{1}"/1 -> netsum/2
  "IW{1,1}"/1("iz{1,1}") -> netsum/1
  Delays 1/1("pd{1,1}") -> "IW{1,1}"/1("pd{1,1}")
  "p{1}"/1 -> Delays 1/1("p{1}")

== system normal/Subsystem1/Function Fitting Neural Network2/Layer 2 ==
  "a{1} " : Inport  PortDimensions=100
      mask Display: e = 0.06;c1 = [120 230 180]/255;c2 = ([120 230 180]+0)/(256+128);c3 = ([120 230 180]+128)/(256+128);patch([0 1 1 0],[0 0 1 1],c1);patch([0 1 1 1-e 1-e 0+e],[0 0 1 1-e 0+e 0+e],c2);patch([0 0 1 1-e 0+e 0+e],[0 1 1 1-e 1-e 0+e],c3);plot([0 1 1 0 0],[0 0 1 1 0]);
  Delays 1 : Subsystem
      mask Display: e = 0.06;c1 = [120 150 230]/255;c2 = ([120 150 230]+0)/383;c3 = ([120 150 230]+128)/383;patch([0 1 1 0],[0 0 1 1],c1);patch([0 1 1 1-e 1-e 0+e],[0 0 1 1-e 0+e 0+e],c2);patch([0 0 1 1-e 0+e 0+e],[0 1 1 1-e 1-e 0+e],c3);plot([0 1 1 0 0],[0 0 1 1 0]);disp('0');
  "LW{2,1}" : Subsystem
      mask Display: e = 0.06;c1 = [120 150 230]/255;c2 = ([120 150 230]+0)/383;c3 = ([120 150 230]+128)/383;patch([0 1 1 0],[0 0 1 1],c1);patch([0 1 1 1-e 1-e 0+e],[0 0 1 1-e 0+e 0+e],c2);patch([0 0 1 1-e 0+e 0+e],[0 1 1 1-e 1-e 0+e],c3);plot([0 1 1 0 0],[0 0 1 1 0]);disp('W');
  "b{2}" : Constant  Value=[-0.363560360916543034992542970940121449530124664306640625;0.94287381051161800460391759770573116838932037353515625;-0.4721310287069091504719153817859478294849395751953125;1.0554594603853464374054738073027692735195159912109375]
      mask Display: e = 0.06;c1 = [120 150 230]/255;c2 = ([120 150 230]+0)/383;c3 = ([120 150 230]+128)/383;patch([0 1 1 0],[0 0 1 1],c1);patch([0 1 1 1-e 1-e 0+e],[0 0 1 1-e 0+e 0+e],c2);patch([0 0 1 1-e 0+e 0+e],[0 1 1 1-e 1-e 0+e],c3);plot([0 1 1 0 0],[0 0 1 1 0]);disp('b');
  netsum : Sum  Inputs=2  InputSameDT=on  SaturateOnIntegerOverflow=on  OutDataTypeStr=Inherit: Same as first input
      mask Display: e = 0.06;c1 = [120 150 230]/255;c2 = ([120 150 230]+0)/383;c3 = ([120 150 230]+128)/383;patch([0 1 1 0],[0 0 1 1],c1);patch([0 1 1 1-e 1-e 0+e],[0 0 1 1-e 0+e 0+e],c2);patch([0 0 1 1-e 0+e 0+e],[0 1 1 1-e 1-e 0+e],c3);plot([0 1 1 0 0],[0 0 1 1 0]);disp('+');
  purelin : neural/Transfer Functions/purelin
  "a{2}" : Outport  InitialOutput=[0;0;0;0]
      mask Display: e = 0.06;c1 = [120 230 180]/255;c2 = ([120 230 180]+0)/(256+128);c3 = ([120 230 180]+128)/(256+128);patch([0 1 1 0],[0 0 1 1],c1);patch([0 1 1 1-e 1-e 0+e],[0 0 1 1-e 0+e 0+e],c2);patch([0 0 1 1-e 0+e 0+e],[0 1 1 1-e 1-e 0+e],c3);plot([0 1 1 0 0],[0 0 1 1 0]);
  wires:
  purelin/1 -> "a{2}"/1
  netsum/1 -> purelin/1
  "b{2}"/1 -> netsum/2
  "LW{2,1}"/1("lz{2,1}") -> netsum/1
  Delays 1/1("pd{2,1}") -> "LW{2,1}"/1("ad{2,1}")
  "a{1} "/1 -> Delays 1/1("p{2}")

== system normal/Subsystem1/Function Fitting Neural Network2/Process Input 1 ==
  x : Inport  PortDimensions=15
      mask Display: e = 0.06;c1 = [120 230 180]/255;c2 = ([120 230 180]+0)/(256+128);c3 = ([120 230 180]+128)/(256+128);patch([0 1 1 0],[0 0 1 1],c1);patch([0 1 1 1-e 1-e 0+e],[0 0 1 1-e 0+e 0+e],c2);patch([0 0 1 1-e 0+e 0+e],[0 1 1 1-e 1-e 0+e],c3);plot([0 1 1 0 0],[0 0 1 1 0]);
  mapminmax : neural/Processing Functions/mapminmax  xmin=[3.97650567133485122184310966986;2.7248060221038734596277208766;4.10876986009723044190877772053;11.7997395123970481023434331291;9.69147739713131528560552396812;3.46457612151836746861022220401;6.39593571872652155718697031261;4.28688363604756350611069137813;6.97687974683904688077973332838;6.4599353632138099001736009086;6.4599353632138099001736009086;1.95063129041178440203907484829;3.49571416389583333739210502245]  xmax=[1771.43499266887192788999527693;1794.0488976631054356403183192;1779.62314843343483516946434975;2484.57589134188310708850622177;2501.74066788909203751245513558;2464.12499617464936818578280509;15623.5974818944614526117220521;15525.5512130097831686725839972;13147.2305966597232327330857515;13696.54294901575485710054636;14757.5569338567456725286319852;4921.13957055568698706338182092;5419.72076307373572490178048611]  ymin=-1  ymax=1
  removeconstantrows : neural/Processing Functions/removeconstantrows  inputSize=15  keep=[1 2 3 4 5 6 7 8 9 11 12 13 15]
      settings: SourceProductBaseCode=NN
  p : Outport  PortDimensions=13
      mask Display: e = 0.06;c1 = [120 230 180]/255;c2 = ([120 230 180]+0)/(256+128);c3 = ([120 230 180]+128)/(256+128);patch([0 1 1 0],[0 0 1 1],c1);patch([0 1 1 1-e 1-e 0+e],[0 0 1 1-e 0+e 0+e],c2);patch([0 0 1 1-e 0+e 0+e],[0 1 1 1-e 1-e 0+e],c3);plot([0 1 1 0 0],[0 0 1 1 0]);
  wires:
  mapminmax/1 -> p/1
  removeconstantrows/1 -> mapminmax/1
  x/1 -> removeconstantrows/1

== system normal/Subsystem1/Function Fitting Neural Network2/Process Output 1 ==
  a : Inport  PortDimensions=4
      mask Display: e = 0.06;c1 = [120 230 180]/255;c2 = ([120 230 180]+0)/(256+128);c3 = ([120 230 180]+128)/(256+128);patch([0 1 1 0],[0 0 1 1],c1);patch([0 1 1 1-e 1-e 0+e],[0 0 1 1-e 0+e 0+e],c2);patch([0 0 1 1-e 0+e 0+e],[0 1 1 1-e 1-e 0+e],c3);plot([0 1 1 0 0],[0 0 1 1 0]);
  mapminmax_reverse : neural/Processing Functions/mapminmax_reverse  xmin=[0;0;0;0]  xmax=[1;1;1;1]  ymin=-1  ymax=1
  y : Outport  PortDimensions=4
      mask Display: e = 0.06;c1 = [120 230 180]/255;c2 = ([120 230 180]+0)/(256+128);c3 = ([120 230 180]+128)/(256+128);patch([0 1 1 0],[0 0 1 1],c1);patch([0 1 1 1-e 1-e 0+e],[0 0 1 1-e 0+e 0+e],c2);patch([0 0 1 1-e 0+e 0+e],[0 1 1 1-e 1-e 0+e],c3);plot([0 1 1 0 0],[0 0 1 1 0]);
  wires:
  mapminmax_reverse/1 -> y/1
  a/1 -> mapminmax_reverse/1

== system normal/Subsystem1/Function Fitting Neural Network/Layer 1/Delays 1 ==
  "p{1}" : Inport  PortDimensions=9
      mask Display: e = 0.06;c1 = [120 230 180]/255;c2 = ([120 230 180]+0)/(256+128);c3 = ([120 230 180]+128)/(256+128);patch([0 1 1 0],[0 0 1 1],c1);patch([0 1 1 1-e 1-e 0+e],[0 0 1 1-e 0+e 0+e],c2);patch([0 0 1 1-e 0+e 0+e],[0 1 1 1-e 1-e 0+e],c3);plot([0 1 1 0 0],[0 0 1 1 0]);
  mux : Mux  Inputs=1
      mask Display: e = 0.06;c1 = [120 150 230]/255;c2 = ([120 150 230]+0)/383;c3 = ([120 150 230]+128)/383;patch([0 1 1 0],[0 0 1 1],c1);patch([0 1 1 1-e 1-e 0+e],[0 0 1 1-e 0+e 0+e],c2);patch([0 0 1 1-e 0+e 0+e],[0 1 1 1-e 1-e 0+e],c3);plot([0 1 1 0 0],[0 0 1 1 0]);disp('Mux')
  "pd{1,1}" : Outport
      mask Display: e = 0.06;c1 = [120 230 180]/255;c2 = ([120 230 180]+0)/(256+128);c3 = ([120 230 180]+128)/(256+128);patch([0 1 1 0],[0 0 1 1],c1);patch([0 1 1 1-e 1-e 0+e],[0 0 1 1-e 0+e 0+e],c2);patch([0 0 1 1-e 0+e 0+e],[0 1 1 1-e 1-e 0+e],c3);plot([0 1 1 0 0],[0 0 1 1 0]);
  wires:
  "p{1}"/1 -> mux/1
  mux/1 -> "pd{1,1}"/1
